simulink model "Autonomous_Driving_Car_Example1"  (R2022a)
settings: Solver=ode2  StartTime=0.0  StopTime=inf  FixedStep=1/600  RelTol=1e-3  EnableMultiTasking=on
model workspace (MAT data in the model file):
  camera_rate : Simulink.Parameter (value not decoded)
  depth_rate : Simulink.Parameter (value not decoded)
symbols that are objects in the model workspace (value not decoded): camera_rate, depth_rate
undefined symbols (not defined in the file): gcbh, height, HIL, JPEG, left, qc_get_step_size, top, Video3D, video_display_show, width
libraries: quarc_library x45, simulink x12
(part 2 of 2)

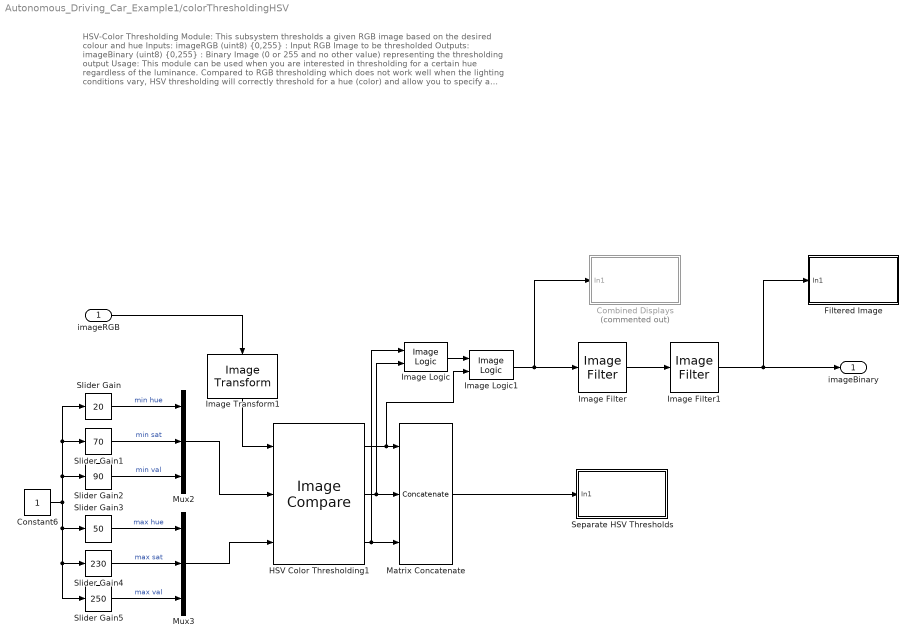
== system Autonomous_Driving_Car_Example1/colorThresholdingHSV ==
  note: HSV-Color Thresholding Module:
      |
      | This subsystem thresholds a given RGB image based on the desired colour and hue
      |
      | Inputs:
      | imageRGB (uint8) {0,255} : Input RGB Image to be thresholded
      |
      | Outputs:
      | imageBinary (uint8) {0,255} : Binary Image (0 or 255 and no other value) representing the thresholding output
      |
      | Usage:
      | This module can be used when you are interested in thresholding for a certain hue regardless of the luminance. Compared to RGB thresholding which does not work well when the lighting conditions vary, HSV thresholding will correctly threshold for a hue (color) and allow you to specify a broad range of illuminance via the saturation and value thresholds.
      |
      | The Separate HSV Thresholds display can help you tune the hue, saturation, and value separately. The final output is the logical and of the three images. The image filter sizes can be used to remove noise (Minimum) and fill holes (Maximum).
  imageRGB : Inport
  Combined Displays : Subsystem  Commented=on  LoadFcn=set_param(gcbh, 'UserData', gcb);  StartFcn=video_display_show([gcb, '/Video Display'], 'add', gcb);  mask(Video Compressed Display){algorithm=JPEG, quality=50, sample_time=-1, use_hardware=on}
      mask prompts: algorithm "Compression algorithm:"; quality "Compression quality (0-100):"; sample_time "Sample time (seconds):"; use_hardware "Use hardware acceleration for video display"
      mask help: Displays a video stream on the host, using compression to minimize bandwidth.
      mask init:
      | qc_set_display('Video\nCompressed\nDisplay');
      settings: UndoDeleteFcn=set_param(gcbh, 'UserData', gcb);  OpenFcn=video_display_show([gcb, '/Video Display'], 'show', gcb);  PreDeleteFcn=video_display_show([gcb, '/Video Display'], 'delete');
      settings: CopyFcn=|
      | set_param(gcbh, 'UserData', gcb);
      | set_param(gcbh, 'LinkStatus', 'none');
      settings: NameChangeFcn=|
      | video_display_show([get_param(gcbh, 'UserData'), '/Video Display'], 'rename', [gcb, '/Video Display']);
      | video_display_show([gcb, '/Video Display'], 'add', gcb);
      | set_param(gcbh, 'UserData', gcb);
      mask Help: web(qc_get_block_help_path(gcb));
      mask TypeOptions algorithm: Image Compress/algorithm
      mask TypeOptions quality: Image Compress/quality
      mask TypeOptions sample_time: Video Display/sample_time
      mask TypeOptions use_hardware: Video Display/use_hardware
      mask Display:
      | patch([0.98591 0.98591 0.62618 0.59072 0.56147   0.536   0.536  0.5441 0.56912 0.59207 0.60881 0.62276 0.63527 0.64364  0.6485  0.6485 0.64706 0.64499 0.63662 0.62411 0.61232 0.59837 0.58307 0.56147   0.536   0.536  0.5441  0.5747 0.60953 0.63662 0.67001  0.7034 0.72851 0.75425 0.77927 0.80294 0.82454 0.84119 0.85865 0.87395 0.88574 0.89339  0.8969 0.89969 0.89969 0.89267  0.8816 0.87044 0.85649  0.8384 0.81824 0.80294 0.78764 0.77513 0.76676 0.75776 0.76397 0.77513 0.79178 0.80987 0.82796 0.84326 0.86207 0.98528],[0.18689 0.05522 0.05522 0.05171 0.05171    0.05 0.18338 0.18338 0.19148 0.20435 0.22298 0.24863 0.28589 0.33125 0.38138 0.55139 0.59801 0.63761 0.68189 0.72149 0.74939 0.76694 0.77855 0.79367 0.79952 0.92768 0.92768 0.92768 0.92417 0.92066 0.91364  0.9032 0.89384 0.88106 0.86594 0.85073 0.82634 0.80537 0.77855 0.74363 0.70403 0.65858 0.61079 0.59099 0.41513 0.37202 0.31847 0.29048 0.25556 0.23342  0.2102 0.19382 0.18221 0.17285 0.16943 0.16124  0.1589 0.16241 0.16709 0.17168  0.1787 0.18221 0.18689 0.18689],[0.9,0.90,0.91])
      | patch([0.536 0.52601 0.46823 0.44528 0.41603 0.39101 0.35555 0.33116 0.31451 0.29291  0.2804 0.26717 0.25322 0.23999 0.22406 0.20732 0.19337 0.17528 0.15935 0.14396 0.13217 0.11759 0.10922 0.10085 0.09671 0.09392 0.09041 0.08906 0.08906 0.09464  0.0995 0.10778 0.11894 0.13145 0.14675 0.16349 0.17672 0.19409 0.20732 0.22406 0.23999 0.26159 0.27833 0.29849 0.31793 0.33602 0.35411 0.37085 0.39245 0.41603   0.536   0.536 0.53159 0.46409   0.446 0.42026 0.39587 0.37571 0.36113 0.34925 0.34088 0.33809 0.33809 0.34088 0.34583 0.35627 0.36392 0.38129 0.39587 0.41117 0.42719 0.44672  0.4676 0.48353 0.48353 0.52394   0.536],[0.05 0.04829 0.04712 0.04712 0.04829 0.05063 0.05405 0.05873 0.06107 0.06692 0.07043 0.07619 0.08087 0.08672 0.09482 0.10652 0.11696 0.13325  0.1508 0.17168 0.19499 0.22415 0.25439 0.28472 0.31379 0.35456 0.38489 0.41513 0.58055 0.63878 0.68774 0.72149 0.75641 0.78089 0.80537 0.82859 0.84029 0.85658 0.86594 0.87404  0.8834 0.89267 0.90086 0.90788 0.91247 0.91832 0.92066   0.923 0.92651 0.92768 0.92768 0.79952 0.79952 0.79952 0.79718 0.78899 0.77153 0.75056 0.72149 0.68072 0.62249  0.5549 0.41396 0.37085 0.33242 0.28121 0.25205 0.22181 0.20552 0.19499 0.18572 0.18221 0.17753 0.17636 0.17753  0.1787  0.1787],[0.9,0.90,0.91])
      | disp('Video\nCompressed\nDisplay');
  Constant6 : Constant
  Filtered Image : Subsystem  LoadFcn=set_param(gcbh, 'UserData', gcb);  StartFcn=video_display_show([gcb, '/Video Display'], 'add', gcb);  mask(Video Compressed Display){algorithm=JPEG, quality=50, sample_time=-1, use_hardware=on}
      mask prompts: algorithm "Compression algorithm:"; quality "Compression quality (0-100):"; sample_time "Sample time (seconds):"; use_hardware "Use hardware acceleration for video display"
      mask help: Displays a video stream on the host, using compression to minimize bandwidth.
      mask init:
      | qc_set_display('Video\nCompressed\nDisplay');
      settings: UndoDeleteFcn=set_param(gcbh, 'UserData', gcb);  OpenFcn=video_display_show([gcb, '/Video Display'], 'show', gcb);  PreDeleteFcn=video_display_show([gcb, '/Video Display'], 'delete');
      settings: CopyFcn=|
      | set_param(gcbh, 'UserData', gcb);
      | set_param(gcbh, 'LinkStatus', 'none');
      settings: NameChangeFcn=|
      | video_display_show([get_param(gcbh, 'UserData'), '/Video Display'], 'rename', [gcb, '/Video Display']);
      | video_display_show([gcb, '/Video Display'], 'add', gcb);
      | set_param(gcbh, 'UserData', gcb);
      mask Help: web(qc_get_block_help_path(gcb));
      mask TypeOptions algorithm: Image Compress/algorithm
      mask TypeOptions quality: Image Compress/quality
      mask TypeOptions sample_time: Video Display/sample_time
      mask TypeOptions use_hardware: Video Display/use_hardware
      mask Display:
      | patch([0.98591 0.98591 0.62618 0.59072 0.56147   0.536   0.536  0.5441 0.56912 0.59207 0.60881 0.62276 0.63527 0.64364  0.6485  0.6485 0.64706 0.64499 0.63662 0.62411 0.61232 0.59837 0.58307 0.56147   0.536   0.536  0.5441  0.5747 0.60953 0.63662 0.67001  0.7034 0.72851 0.75425 0.77927 0.80294 0.82454 0.84119 0.85865 0.87395 0.88574 0.89339  0.8969 0.89969 0.89969 0.89267  0.8816 0.87044 0.85649  0.8384 0.81824 0.80294 0.78764 0.77513 0.76676 0.75776 0.76397 0.77513 0.79178 0.80987 0.82796 0.84326 0.86207 0.98528],[0.18689 0.05522 0.05522 0.05171 0.05171    0.05 0.18338 0.18338 0.19148 0.20435 0.22298 0.24863 0.28589 0.33125 0.38138 0.55139 0.59801 0.63761 0.68189 0.72149 0.74939 0.76694 0.77855 0.79367 0.79952 0.92768 0.92768 0.92768 0.92417 0.92066 0.91364  0.9032 0.89384 0.88106 0.86594 0.85073 0.82634 0.80537 0.77855 0.74363 0.70403 0.65858 0.61079 0.59099 0.41513 0.37202 0.31847 0.29048 0.25556 0.23342  0.2102 0.19382 0.18221 0.17285 0.16943 0.16124  0.1589 0.16241 0.16709 0.17168  0.1787 0.18221 0.18689 0.18689],[0.9,0.90,0.91])
      | patch([0.536 0.52601 0.46823 0.44528 0.41603 0.39101 0.35555 0.33116 0.31451 0.29291  0.2804 0.26717 0.25322 0.23999 0.22406 0.20732 0.19337 0.17528 0.15935 0.14396 0.13217 0.11759 0.10922 0.10085 0.09671 0.09392 0.09041 0.08906 0.08906 0.09464  0.0995 0.10778 0.11894 0.13145 0.14675 0.16349 0.17672 0.19409 0.20732 0.22406 0.23999 0.26159 0.27833 0.29849 0.31793 0.33602 0.35411 0.37085 0.39245 0.41603   0.536   0.536 0.53159 0.46409   0.446 0.42026 0.39587 0.37571 0.36113 0.34925 0.34088 0.33809 0.33809 0.34088 0.34583 0.35627 0.36392 0.38129 0.39587 0.41117 0.42719 0.44672  0.4676 0.48353 0.48353 0.52394   0.536],[0.05 0.04829 0.04712 0.04712 0.04829 0.05063 0.05405 0.05873 0.06107 0.06692 0.07043 0.07619 0.08087 0.08672 0.09482 0.10652 0.11696 0.13325  0.1508 0.17168 0.19499 0.22415 0.25439 0.28472 0.31379 0.35456 0.38489 0.41513 0.58055 0.63878 0.68774 0.72149 0.75641 0.78089 0.80537 0.82859 0.84029 0.85658 0.86594 0.87404  0.8834 0.89267 0.90086 0.90788 0.91247 0.91832 0.92066   0.923 0.92651 0.92768 0.92768 0.79952 0.79952 0.79952 0.79718 0.78899 0.77153 0.75056 0.72149 0.68072 0.62249  0.5549 0.41396 0.37085 0.33242 0.28121 0.25205 0.22181 0.20552 0.19499 0.18572 0.18221 0.17753 0.17636 0.17753  0.1787  0.1787],[0.9,0.90,0.91])
      | disp('Video\nCompressed\nDisplay');
  HSV Color Thresholding1 : quarc_library/Image Processing/Generic/Image Compare  output_type=Separate planes (three HxW outputs)  source=External input ports  r_comparison=min <= pixel and pixel <= max with wrapping  r_minimum=30  r_maximum=70  g_comparison=min <= pixel and pixel <= max  g_minimum=60  g_maximum=100  b_comparison=min <= pixel and pixel <= max  b_minimum=40  b_maximum=80
      settings: SourceProductName=QUARC Targets
  Image Filter : quarc_library/Image Processing/Generic/Image Filter  filter_type=Minimum  source_of_roi=Internal dialog parameter  roi_style=[top, left, height, width]  roi=[]  maximum_roi=[]  roi_zone=Operate inside region of interest  border_type=Replicate  border_value=[0 0 0]  kernel_size=5  sigma=10  mask_size=[3 3]  kernel=int16([-2 -1 0; -1 1 1; 0 1 2])  divisor=1  offset=0  rounding=Nearest  algorithm_hint=None  threshold=100  alpha=0.9  num_frames=8  num_valid=1  gap_threshold=10  depth_threshold=255  iterations=2
      settings: AttributesFormatString=(%<filter_type>)  SourceProductName=QUARC Targets
  Image Filter1 : quarc_library/Image Processing/Generic/Image Filter  filter_type=Maximum  source_of_roi=Internal dialog parameter  roi_style=[top, left, height, width]  roi=[]  maximum_roi=[]  roi_zone=Operate inside region of interest  border_type=Replicate  border_value=[0 0 0]  kernel_size=5  sigma=10  mask_size=[7 7]  kernel=int16([-2 -1 0; -1 1 1; 0 1 2])  divisor=1  offset=0  rounding=Nearest  algorithm_hint=None  threshold=100  alpha=0.9  num_frames=8  num_valid=1  gap_threshold=10  depth_threshold=255  iterations=2
      settings: AttributesFormatString=(%<filter_type>)  SourceProductName=QUARC Targets
  Image Logic : quarc_library/Image Processing/Generic/Image Logic  algorithm=AND  source=Internal dialog parameter  row=0  column=0
      settings: AttributesFormatString=(%<algorithm>)  SourceProductName=QUARC Targets
  Image Logic1 : quarc_library/Image Processing/Generic/Image Logic  algorithm=AND  source=Internal dialog parameter  row=0  column=0
      settings: AttributesFormatString=(%<algorithm>)  SourceProductName=QUARC Targets
  Image Transform1 : quarc_library/Image Processing/Generic/Image Transform  algorithm=RGB to HSV  color_theme=KRYGCBMW  min_pixel=0  max_pixel=4000  focal_length=308  principal_point=[262 334]  radial_coeffs=[-0.3129 0.0907]  tangential_coeffs=[]  extrapolated_pixel=0  interpolation=nearest  row_coords=0  column_coords=0  output_height=480  output_width=640  angle=0  origin=[240 320]  output_origin=[240 320]  output_data_type=uint8
      settings: AttributesFormatString=(%<algorithm>)  SourceProductName=QUARC Targets
  Matrix Concatenate : Concatenate  NumInputs=3  Mode=Multidimensional array  ConcatenateDimension=2
  Mux2 : Mux  Inputs=3
  Mux3 : Mux  Inputs=3
  Separate HSV Thresholds : Subsystem  LoadFcn=set_param(gcbh, 'UserData', gcb);  StartFcn=video_display_show([gcb, '/Video Display'], 'add', gcb);  mask(Video Compressed Display){algorithm=JPEG, quality=50, sample_time=-1, use_hardware=on}
      mask prompts: algorithm "Compression algorithm:"; quality "Compression quality (0-100):"; sample_time "Sample time (seconds):"; use_hardware "Use hardware acceleration for video display"
      mask help: Displays a video stream on the host, using compression to minimize bandwidth.
      mask init:
      | qc_set_display('Video\nCompressed\nDisplay');
      settings: UndoDeleteFcn=set_param(gcbh, 'UserData', gcb);  OpenFcn=video_display_show([gcb, '/Video Display'], 'show', gcb);  PreDeleteFcn=video_display_show([gcb, '/Video Display'], 'delete');
      settings: CopyFcn=|
      | set_param(gcbh, 'UserData', gcb);
      | set_param(gcbh, 'LinkStatus', 'none');
      settings: NameChangeFcn=|
      | video_display_show([get_param(gcbh, 'UserData'), '/Video Display'], 'rename', [gcb, '/Video Display']);
      | video_display_show([gcb, '/Video Display'], 'add', gcb);
      | set_param(gcbh, 'UserData', gcb);
      mask Help: web(qc_get_block_help_path(gcb));
      mask TypeOptions algorithm: Image Compress/algorithm
      mask TypeOptions quality: Image Compress/quality
      mask TypeOptions sample_time: Video Display/sample_time
      mask TypeOptions use_hardware: Video Display/use_hardware
      mask Display:
      | patch([0.98591 0.98591 0.62618 0.59072 0.56147   0.536   0.536  0.5441 0.56912 0.59207 0.60881 0.62276 0.63527 0.64364  0.6485  0.6485 0.64706 0.64499 0.63662 0.62411 0.61232 0.59837 0.58307 0.56147   0.536   0.536  0.5441  0.5747 0.60953 0.63662 0.67001  0.7034 0.72851 0.75425 0.77927 0.80294 0.82454 0.84119 0.85865 0.87395 0.88574 0.89339  0.8969 0.89969 0.89969 0.89267  0.8816 0.87044 0.85649  0.8384 0.81824 0.80294 0.78764 0.77513 0.76676 0.75776 0.76397 0.77513 0.79178 0.80987 0.82796 0.84326 0.86207 0.98528],[0.18689 0.05522 0.05522 0.05171 0.05171    0.05 0.18338 0.18338 0.19148 0.20435 0.22298 0.24863 0.28589 0.33125 0.38138 0.55139 0.59801 0.63761 0.68189 0.72149 0.74939 0.76694 0.77855 0.79367 0.79952 0.92768 0.92768 0.92768 0.92417 0.92066 0.91364  0.9032 0.89384 0.88106 0.86594 0.85073 0.82634 0.80537 0.77855 0.74363 0.70403 0.65858 0.61079 0.59099 0.41513 0.37202 0.31847 0.29048 0.25556 0.23342  0.2102 0.19382 0.18221 0.17285 0.16943 0.16124  0.1589 0.16241 0.16709 0.17168  0.1787 0.18221 0.18689 0.18689],[0.9,0.90,0.91])
      | patch([0.536 0.52601 0.46823 0.44528 0.41603 0.39101 0.35555 0.33116 0.31451 0.29291  0.2804 0.26717 0.25322 0.23999 0.22406 0.20732 0.19337 0.17528 0.15935 0.14396 0.13217 0.11759 0.10922 0.10085 0.09671 0.09392 0.09041 0.08906 0.08906 0.09464  0.0995 0.10778 0.11894 0.13145 0.14675 0.16349 0.17672 0.19409 0.20732 0.22406 0.23999 0.26159 0.27833 0.29849 0.31793 0.33602 0.35411 0.37085 0.39245 0.41603   0.536   0.536 0.53159 0.46409   0.446 0.42026 0.39587 0.37571 0.36113 0.34925 0.34088 0.33809 0.33809 0.34088 0.34583 0.35627 0.36392 0.38129 0.39587 0.41117 0.42719 0.44672  0.4676 0.48353 0.48353 0.52394   0.536],[0.05 0.04829 0.04712 0.04712 0.04829 0.05063 0.05405 0.05873 0.06107 0.06692 0.07043 0.07619 0.08087 0.08672 0.09482 0.10652 0.11696 0.13325  0.1508 0.17168 0.19499 0.22415 0.25439 0.28472 0.31379 0.35456 0.38489 0.41513 0.58055 0.63878 0.68774 0.72149 0.75641 0.78089 0.80537 0.82859 0.84029 0.85658 0.86594 0.87404  0.8834 0.89267 0.90086 0.90788 0.91247 0.91832 0.92066   0.923 0.92651 0.92768 0.92768 0.79952 0.79952 0.79952 0.79718 0.78899 0.77153 0.75056 0.72149 0.68072 0.62249  0.5549 0.41396 0.37085 0.33242 0.28121 0.25205 0.22181 0.20552 0.19499 0.18572 0.18221 0.17753 0.17636 0.17753  0.1787  0.1787],[0.9,0.90,0.91])
      | disp('Video\nCompressed\nDisplay');
  Slider Gain : simulink/Math Operations/Slider Gain  gain=20  low=0  high=255
  Slider Gain1 : simulink/Math Operations/Slider Gain  gain=70  low=0  high=255
  Slider Gain2 : simulink/Math Operations/Slider Gain  gain=90  low=0  high=255
  Slider Gain3 : simulink/Math Operations/Slider Gain  gain=50  low=0  high=255
  Slider Gain4 : simulink/Math Operations/Slider Gain  gain=230  low=0  high=255
  Slider Gain5 : simulink/Math Operations/Slider Gain  gain=250  low=0  high=255
  imageBinary : Outport  VectorParamsAs1DForOutWhenUnconnected=off
  wires:
  HSV Color Thresholding1/3 -> Image Logic/1, Matrix Concatenate/3
  Image Logic1/1 -> Combined Displays/1(In1), Image Filter/1
  Image Logic/1 -> Image Logic1/1
  Matrix Concatenate/1 -> Separate HSV Thresholds/1(In1)
  Mux2/1 -> HSV Color Thresholding1/2
  Image Transform1/1 -> HSV Color Thresholding1/1
  Slider Gain/1 -> Mux2/1  "min hue"
  HSV Color Thresholding1/2 -> Image Logic/2, Matrix Concatenate/2
  Slider Gain5/1 -> Mux3/3  "max val"
  Slider Gain2/1 -> Mux2/3  "min val"
  Mux3/1 -> HSV Color Thresholding1/3
  Slider Gain1/1 -> Mux2/2  "min sat"
  Slider Gain4/1 -> Mux3/2  "max sat"
  HSV Color Thresholding1/1 -> Image Logic1/2, Matrix Concatenate/1
  Constant6/1 -> Slider Gain/1, Slider Gain1/1, Slider Gain2/1, Slider Gain3/1, Slider Gain5/1, Slider Gain4/1
  imageRGB/1 -> Image Transform1/1
  Slider Gain3/1 -> Mux3/1  "max hue"
  Image Filter/1 -> Image Filter1/1
  Image Filter1/1 -> Filtered Image/1(In1), imageBinary/1

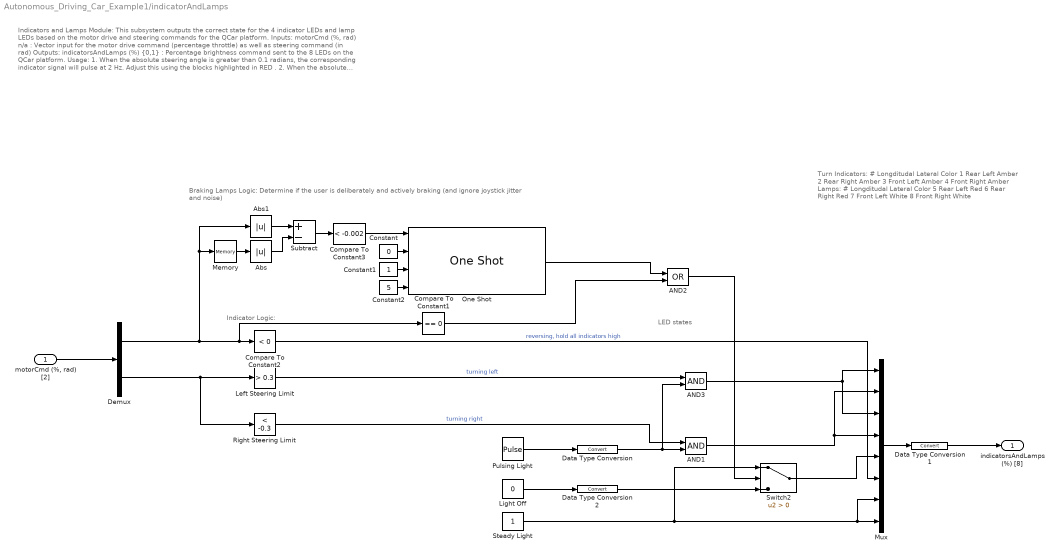
== system Autonomous_Driving_Car_Example1/indicatorAndLamps ==
  note: Indicators and Lamps Module:
      |
      | This subsystem outputs the correct state for the 4 indicator LEDs and lamp LEDs based on the motor drive and steering commands for the QCar platform.
      |
      | Inputs:
      | motorCmd (%, rad) n/a : Vector input for the motor drive command (percentage throttle) as well as steering command (in rad)
      |
      | Outputs:
      | indicatorsAndLamps (%) {0,1} : Percentage brightness command sent to the 8 LEDs on the QCar platform.
      |
      | Usage:
      | 1. When the absolute steering angle is greater than 0.1 radians, the corresponding indicator signal will pulse at 2 Hz. Adjust this using the blocks highlighted in RED .
      | 2. When the absolute motor drive command approaches 0, the brake lamps will receive 100% brightness command, and 0% brightness otherwise. Adjust this using the blocks highlighted in GREEN .
  note: Braking Lamps Logic:
      | Determine if the user is deliberately and actively braking (and ignore joystick jitter and noise)
  note: LED states
  note: Turn Indicators:
      | # Longditudal Lateral Color
      | 1 Rear Left Amber
      | 2 Rear Right Amber
      | 3 Front Left Amber
      | 4 Front Right Amber
      |
      | Lamps:
      | # Longditudal Lateral Color
      | 5 Rear Left Red
      | 6 Rear Right Red
      | 7 Front Left White
      | 8 Front Right White
  note: Indicator Logic:
  "motorCmd (%, rad) [2]" : Inport
  AND1 : Logic  IconShape=distinctive  AllPortsSameDT=off  OutDataTypeStr=boolean
  AND2 : Logic  Operator=OR  IconShape=distinctive  AllPortsSameDT=off  OutDataTypeStr=boolean
  AND3 : Logic  IconShape=distinctive  AllPortsSameDT=off  OutDataTypeStr=boolean
  Abs : Abs  SaturateOnIntegerOverflow=off
  Abs1 : Abs  SaturateOnIntegerOverflow=off
  Compare To Constant1 : simulink/Logic and Bit Operations/Compare To Constant  relop===  const=0  OutDataTypeStr=uint8
  Compare To Constant2 : simulink/Logic and Bit Operations/Compare To Constant  relop=<  const=0  OutDataTypeStr=boolean
  Compare To Constant3 : simulink/Logic and Bit Operations/Compare To Constant  relop=<  const=-0.002  OutDataTypeStr=boolean
  Constant : Constant  Value=0
  Constant1 : Constant
  Constant2 : Constant  Value=5
  Data Type Conversion : DataTypeConversion  SaturateOnIntegerOverflow=off  RndMeth=Floor
  Data Type Conversion1 : DataTypeConversion  SaturateOnIntegerOverflow=off  RndMeth=Floor
  Data Type Conversion2 : DataTypeConversion  SaturateOnIntegerOverflow=off  RndMeth=Floor
  Demux : Demux  Outputs=2
  Left Steering Limit : simulink/Logic and Bit Operations/Compare To Constant  relop=>  const=0.3  OutDataTypeStr=boolean
  Light Off : Constant  Value=0  OutDataTypeStr=boolean
  Memory : Memory
  Mux : Mux  Inputs=8
  One Shot : quarc_library/Discontinuities/One Shot  trigger_type=Falling edge  redun_pulse=Ignore extraneous pulse  width_source=External input port  pulse_width=100
      settings: SourceProductName=QUARC Targets
  Pulsing Light : DiscretePulseGenerator  Period=0.5/qc_get_step_size  PulseWidth=0.5/2/qc_get_step_size  SampleTime=qc_get_step_size
  Right Steering Limit : simulink/Logic and Bit Operations/Compare To Constant  relop=<  const=-0.3  OutDataTypeStr=boolean
  Steady Light : Constant  OutDataTypeStr=boolean
  Subtract : Sum  Inputs=+-
  Switch2 : Switch  Criteria=u2 > Threshold  SaturateOnIntegerOverflow=off  InputSameDT=off
  indicatorsAndLamps (%) [8] : Outport  VectorParamsAs1DForOutWhenUnconnected=off
  wires:
  Data Type Conversion2/1 -> Switch2/3
  Demux/2 -> Right Steering Limit/1, Left Steering Limit/1
  Light Off/1 -> Data Type Conversion2/1
  One Shot/1 -> AND2/1
  Steady Light/1 -> Mux/7, Mux/8, Switch2/1
  Compare To Constant3/1 -> One Shot/1
  Constant2/1 -> One Shot/4
  Right Steering Limit/1 -> AND1/1  "turning right"
  Mux/1 -> Data Type Conversion1/1
  Constant/1 -> One Shot/2
  Pulsing Light/1 -> Data Type Conversion/1
  Abs/1 -> Subtract/2
  Memory/1 -> Abs/1
  Abs1/1 -> Subtract/1
  Data Type Conversion/1 -> AND3/2, AND1/2
  Data Type Conversion1/1 -> indicatorsAndLamps (%) [8]/1
  Left Steering Limit/1 -> AND3/1  "turning left"
  Switch2/1 -> Mux/5
  Constant1/1 -> One Shot/3
  Demux/1 -> Compare To Constant1/1, Compare To Constant2/1, Memory/1, Abs1/1
  AND3/1 -> Mux/1, Mux/3
  "motorCmd (%, rad) [2]"/1 -> Demux/1
  Subtract/1 -> Compare To Constant3/1
  AND1/1 -> Mux/2, Mux/4
  Compare To Constant2/1 -> Mux/6  "reversing, hold all indicators high"
  Compare To Constant1/1 -> AND2/2
  AND2/1 -> Switch2/2

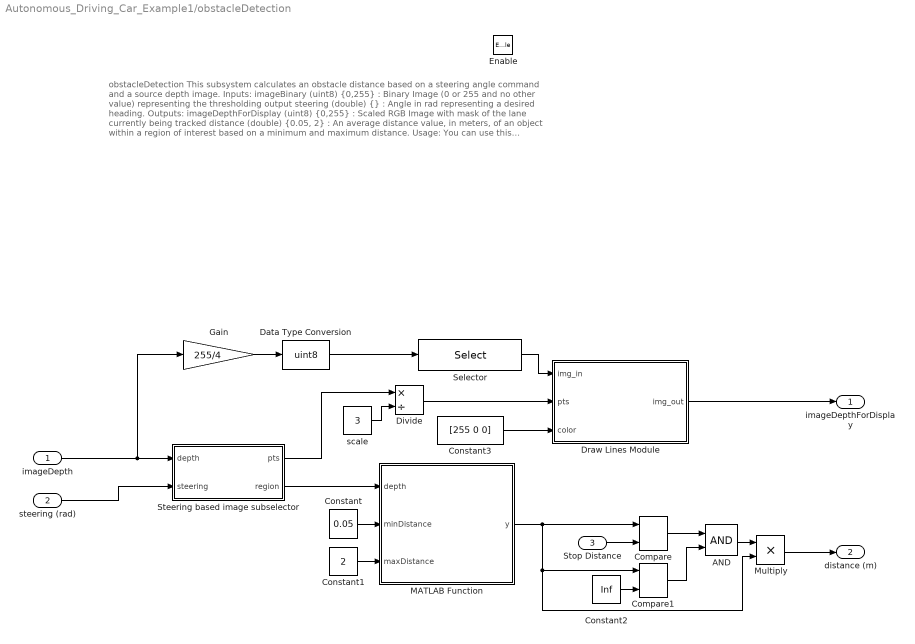
== system Autonomous_Driving_Car_Example1/obstacleDetection ==
  note: obstacleDetection
      | This subsystem calculates an obstacle distance based on a steering angle command and a source depth image.
      |
      | Inputs:
      | imageBinary (uint8) {0,255} : Binary Image (0 or 255 and no other value) representing the thresholding output
      | steering (double) {} : Angle in rad representing a desired heading.
      |
      | Outputs:
      | imageDepthForDisplay (uint8) {0,255} : Scaled RGB Image with mask of the lane currently being tracked
      | distance (double) {0.05, 2} : An average distance value, in meters, of an object within a region of interest based on a minimum and maximum distance.
      |
      | Usage:
      |
      | You can use this subsystem to determine if the desired heading angle will cause the car to colllide with an obstacle by examining the distances from a region of interest within the depth image and calculating how far the obstacle is.
  imageDepth : Inport
  steering (rad) : Inport  Port=2
  Stop Distance : Inport  Port=3
  Enable : EnablePort  PropagateVarSize=During execution
  AND : Logic  AllPortsSameDT=off  OutDataTypeStr=boolean
  Compare : quarc_library/Logic Operations/Compare  operator=>=  output_data_type=boolean
      settings: SourceProductName=QUARC Targets
  Compare1 : quarc_library/Logic Operations/Compare  operator=<  output_data_type=boolean
      settings: SourceProductName=QUARC Targets
  Constant : Constant  Value=0.05
  Constant1 : Constant  Value=2
  Constant2 : Constant  Value=Inf
  Constant3 : Constant  Value=[255 0 0]
  Data Type Conversion : DataTypeConversion  OutDataTypeStr=uint8  SaturateOnIntegerOverflow=off  RndMeth=Floor
  Divide : Product  Inputs=*/  OutDataTypeStr=Inherit: Inherit via back propagation
  Draw Lines Module : MATLAB Function  TreatAsAtomicUnit=on
  Gain : Gain  Gain=255/4
  MATLAB Function : MATLAB Function  TreatAsAtomicUnit=on
  Multiply : Product
  Selector : Selector  NumberOfDimensions=2  InputPortWidth=3  IndexOptions=Index vector (dialog),Index vector (dialog)  Indices=[1:3:360],[1:3:640]  OutputSizes=1,1
  Steering based image subselector : MATLAB Function  TreatAsAtomicUnit=on
  scale : Constant  Value=3
  imageDepthForDisplay : Outport  VectorParamsAs1DForOutWhenUnconnected=off
  distance (m) : Outport  Port=2  VectorParamsAs1DForOutWhenUnconnected=off
  wires:
  Constant3/1 -> Draw Lines Module/3(color)
  Steering based image subselector/1(pts) -> Divide/1
  Steering based image subselector/2(region) -> MATLAB Function/1(depth)
  steering (rad)/1 -> Steering based image subselector/2(steering)
  Multiply/1 -> distance (m)/1
  Constant1/1 -> MATLAB Function/3(maxDistance)
  Constant/1 -> MATLAB Function/2(minDistance)
  MATLAB Function/1(y) -> Compare/1, Multiply/2, Compare1/1
  imageDepth/1 -> Steering based image subselector/1(depth), Gain/1
  Selector/1 -> Draw Lines Module/1(img_in)
  Data Type Conversion/1 -> Selector/1
  Divide/1 -> Draw Lines Module/2(pts)
  Draw Lines Module/1(img_out) -> imageDepthForDisplay/1
  scale/1 -> Divide/2
  Gain/1 -> Data Type Conversion/1
  Stop Distance/1 -> Compare/2
  Compare/1 -> AND/1
  Compare1/1 -> AND/2
  Constant2/1 -> Compare1/2
  AND/1 -> Multiply/1

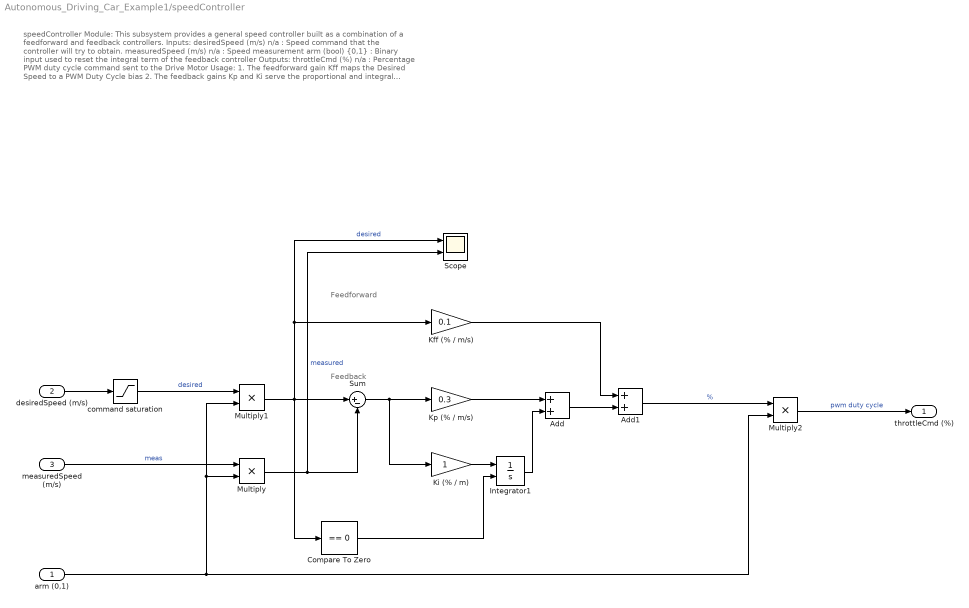
== system Autonomous_Driving_Car_Example1/speedController ==
  note: Feedforward
  note: Feedback
  note: speedController Module:
      |
      | This subsystem provides a general speed controller built as a combination of a feedforward and feedback controllers.
      |
      | Inputs:
      | desiredSpeed (m/s) n/a : Speed command that the controller will try to obtain.
      | measuredSpeed (m/s) n/a : Speed measurement
      | arm (bool) {0,1} : Binary input used to reset the integral term of the feedback controller
      |
      | Outputs:
      | throttleCmd (%) n/a : Percentage PWM duty cycle command sent to the Drive Motor
      |
      | Usage:
      | 1. The feedforward gain Kff maps the Desired Speed to a PWM Duty Cycle bias
      | 2. The feedback gains Kp and Ki serve the proportional and integral terms to output corrections to the PWM Duty Cycle so as to regulate the desired speed.
  arm (0,1) : Inport
  desiredSpeed (m/s) : Inport  Port=2
  measuredSpeed (m/s) : Inport  Port=3
  Add : Sum
  Add1 : Sum
  Compare To Zero : simulink/Logic and Bit Operations/Compare To Zero  relop===  OutDataTypeStr=boolean
  Integrator1 : Integrator  ExternalReset=either  LimitOutput=on  UpperSaturationLimit=0.4  LowerSaturationLimit=-0.4
  Kff (% / m/s) : Gain  Gain=0.1
  "Ki (% / m) " : Gain
  Kp (% / m/s) : Gain  Gain=0.3
  Multiply : Product
  Multiply1 : Product
  Multiply2 : Product
  Scope : Scope  NumInputPorts=2
  Sum : Sum  Inputs=|+-
  command saturation : Saturate  UpperLimit=5  LowerLimit=-5
  throttleCmd (%) : Outport  VectorParamsAs1DForOutWhenUnconnected=off
  wires:
  command saturation/1 -> Multiply1/1  "desired"
  arm (0,1)/1 -> Multiply1/2, Multiply/2, Multiply2/2
  measuredSpeed (m/s)/1 -> Multiply/1  "meas"
  Multiply/1 -> Sum/2, Scope/2  "measured"
  Add/1 -> Add1/2
  Add1/1 -> Multiply2/1  "%"
  Multiply1/1 -> Compare To Zero/1, Sum/1, Kff (% / m/s)/1, Scope/1  "desired"
  Integrator1/1 -> Add/2
  Multiply2/1 -> throttleCmd (%)/1  "pwm duty cycle"
  Kp (% / m/s)/1 -> Add/1
  Compare To Zero/1 -> Integrator1/2
  Kff (% / m/s)/1 -> Add1/1
  Sum/1 -> "Ki (% / m) "/1, Kp (% / m/s)/1
  "Ki (% / m) "/1 -> Integrator1/1
  desiredSpeed (m/s)/1 -> command saturation/1

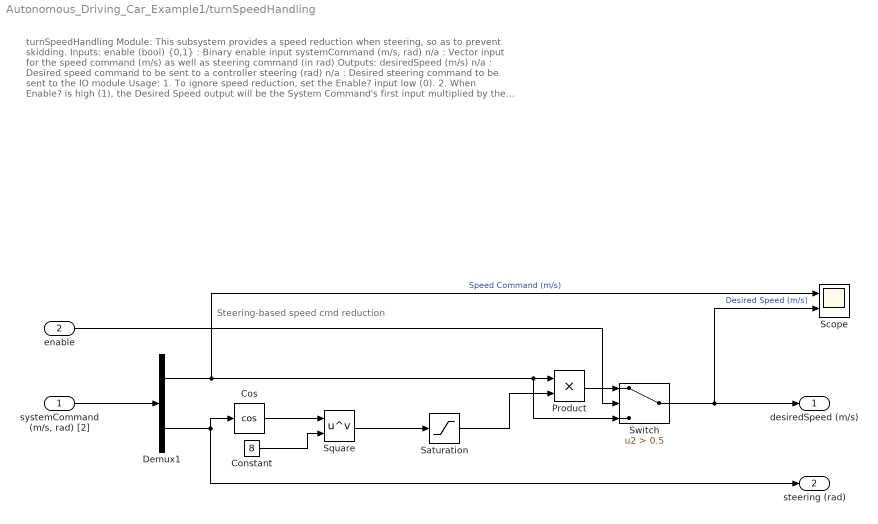
== system Autonomous_Driving_Car_Example1/turnSpeedHandling ==
  note: turnSpeedHandling Module:
      |
      | This subsystem provides a speed reduction when steering, so as to prevent skidding.
      |
      | Inputs:
      | enable (bool) {0,1} : Binary enable input
      | systemCommand (m/s, rad) n/a : Vector input for the speed command (m/s) as well as steering command (in rad)
      |
      | Outputs:
      | desiredSpeed (m/s) n/a : Desired speed command to be sent to a controller
      | steering (rad) n/a : Desired steering command to be sent to the IO module
      |
      | Usage:
      | 1. To ignore speed reduction, set the Enable? input low (0).
      | 2. When Enable? is high (1), the Desired Speed output will be the System Command's first input multiplied by the cosine of the steering. Note that the lower limit of this reduction is set to 50% of the speed command input.
  note: Steering-based speed cmd reduction
  "systemCommand (m/s, rad) [2]" : Inport
  enable : Inport  Port=2
  Constant : Constant  Value=8
  Cos : Trigonometry  Operator=cos
  Demux1 : Demux  Outputs=2
  Product : Product
  Saturation : Saturate  UpperLimit=1  LowerLimit=0.5
  Scope : Scope  NumInputPorts=2
  Square : Math  Operator=pow  SignedPower=on
  Switch : Switch  Criteria=u2 > Threshold  Threshold=0.5  SaturateOnIntegerOverflow=off  InputSameDT=off
  desiredSpeed (m/s) : Outport  VectorParamsAs1DForOutWhenUnconnected=off
  steering (rad) : Outport  Port=2  VectorParamsAs1DForOutWhenUnconnected=off
  wires:
  Cos/1 -> Square/1
  Switch/1 -> desiredSpeed (m/s)/1, Scope/2  "Desired Speed (m/s)"
  Product/1 -> Switch/1
  Saturation/1 -> Product/2
  Demux1/1 -> Product/1, Switch/3, Scope/1  "Speed Command (m/s)"
  "systemCommand (m/s, rad) [2]"/1 -> Demux1/1
  enable/1 -> Switch/2
  Constant/1 -> Square/2
  Demux1/2 -> steering (rad)/1, Cos/1
  Square/1 -> Saturation/1

== system Autonomous_Driving_Car_Example1/colorThresholdingHSV/Combined Displays ==
  In1 : Inport
  Channel : quarc_library/Signal Routing/Channel  channel=2  buffer_size=1
  Image Compress : quarc_library/Image Processing/Generic/Image Compress  algorithm=JPEG  source=Internal dialog parameter  quality=quality  output_dim=-1
  Video Display : quarc_library/Multimedia/Video Display  Tag="Autonomous_Driving_Car_Example1/colorThresholdingHSV/Combined  Displays/Video Display"  sample_time=sample_time  use_hardware=on
  wires:
  Image Compress/1 -> Channel/1
  In1/1 -> Image Compress/1
  Channel/1 -> Video Display/1

== system Autonomous_Driving_Car_Example1/colorThresholdingHSV/Filtered Image ==
  In1 : Inport
  Channel : quarc_library/Signal Routing/Channel  channel=2  buffer_size=1
  Image Compress : quarc_library/Image Processing/Generic/Image Compress  algorithm=JPEG  source=Internal dialog parameter  quality=quality  output_dim=-1
  Video Display : quarc_library/Multimedia/Video Display  Tag=Autonomous_Driving_Car_Example1/colorThresholdingHSV/Filtered Image/Video Display  sample_time=sample_time  use_hardware=on
  wires:
  Image Compress/1 -> Channel/1
  In1/1 -> Image Compress/1
  Channel/1 -> Video Display/1

== system Autonomous_Driving_Car_Example1/colorThresholdingHSV/Separate HSV Thresholds ==
  In1 : Inport
  Channel : quarc_library/Signal Routing/Channel  channel=3  buffer_size=1
  Image Compress : quarc_library/Image Processing/Generic/Image Compress  algorithm=JPEG  source=Internal dialog parameter  quality=quality  output_dim=-1
  Video Display : quarc_library/Multimedia/Video Display  Tag=Autonomous_Driving_Car_Example1/colorThresholdingHSV/Separate HSV Thresholds/Video Display  sample_time=sample_time  use_hardware=on
  wires:
  Channel/1 -> Video Display/1
  In1/1 -> Image Compress/1
  Image Compress/1 -> Channel/1

== matlab function Autonomous_Driving_Car_Example1/ROI Mask/Mask ==
  data: box input; y output
function y = fcn(box)

x_min = box(1);
x_max = box(2);
y_min = box(3);
y_max = box(4);

y = uint8(zeros(200, 820));

y(y_min:y_max, x_min:x_max) = uint8(255);

== matlab function Autonomous_Driving_Car_Example1/Lane Location/MATLAB Function ==
  data: NumberOfObjects input; u input size=2; location output; reference input
function location = fcn(NumberOfObjects, u, reference)

persistent last_location;

location = single([0; 0]);

if isempty(last_location)
    last_location = single([reference; 0]);
end

if NumberOfObjects > 0
    last_location = single([u(1); u(2)]);
end

location = last_location;

== matlab function Autonomous_Driving_Car_Example1/Diagnostics/MATLAB Function3 ==
  data: target input; y output
function y = fcn(target)


% image swaps x and y
y = [1 target(2); 
     410 target(2)];

== matlab function Autonomous_Driving_Car_Example1/Diagnostics/Draw Lines Module2 ==
  data: img_in input; img_out output; pts input; color input
function img_out = drawLines(img_in, pts, color)

% Draw lines connecting the points using the provided color

% Inputs:
% img_in    : Input RGB Image (size = m by n)
% pts       : p x-y pairs of points (px) where markers are to be drawn
% color     : 1x3 matrix of RGB color values for each marker

% Outputs:
% img_out   : Output RGB Image with the markers drawn in (size = m by n)

%% Initialization
if size(img_in, 3) == 3
    img_out = img_in;
elseif size(img_in, 3) == 1
    img_out = cat(3, img_in, img_in, img_in);
end

[p, ~] = size(pts); % determine the number of points

%% Draw the lines
    for i = 1:p-1
        % determine the max(rows_difference, col_difference) between two
        % points
        itr = max(abs(pts(i,1) - pts(i+1,1)), abs(pts(i,2) - pts(i+1,2)));
        
        % generate linear spaces of row and col values between the pts
        row_vec = round(linspace(pts(i,1), pts(i+1,1), itr));
        col_vec = round(linspace(pts(i,2), pts(i+1,2), itr));
        
        % iterate through the values and shade them right

        for j = 1:itr
            img_out(row_vec(j), col_vec(j),1) = color(1);
            img_out(row_vec(j), col_vec(j),2) = color(2);
            img_out(row_vec(j), col_vec(j),3) = color(3);
        end
    end
end

== matlab function Autonomous_Driving_Car_Example1/obstacleDetection/Draw Lines Module ==
  data: img_in input; img_out output; pts input; color input
function img_out = drawLines(img_in, pts, color)

% Draw lines connecting the points using the provided color

% Inputs:
% img_in    : Input RGB Image (size = m by n)
% pts       : p x-y pairs of points (px) where markers are to be drawn
% color     : 1x3 matrix of RGB color values for each marker

% Outputs:
% img_out   : Output RGB Image with the markers drawn in (size = m by n)

%% Initialization
if size(img_in, 3) == 3
    img_out = img_in;
elseif size(img_in, 3) == 1
    img_out = cat(3, img_in, img_in, img_in);
end

[p, ~] = size(pts); % determine the number of points

%% Draw the lines
    for i = 1:p-1
        % determine the max(rows_difference, col_difference) between two
        % points
        itr = max(abs(pts(i,1) - pts(i+1,1)), abs(pts(i,2) - pts(i+1,2)));
        
        % generate linear spaces of row and col values between the pts
        row_vec = round(linspace(pts(i,1), pts(i+1,1), itr));
        col_vec = round(linspace(pts(i,2), pts(i+1,2), itr));
        
        % iterate through the values and shade them right

        for j = 1:itr
            img_out(row_vec(j), col_vec(j),1) = color(1);
            img_out(row_vec(j), col_vec(j),2) = color(2);
            img_out(row_vec(j), col_vec(j),3) = color(3);
        end
    end
end

== matlab function Autonomous_Driving_Car_Example1/MATLAB Function ==
  data: u input; y output
function y = fcn(u)

y = u(211:410,:,:);

== matlab function Autonomous_Driving_Car_Example1/Obstacle_Avoidance ==
  data: obstacle_dist input; target_lane output; current_state output
function [target_lane, current_state] = Obstacle_Avoidance(obstacle_dist)
% Ground-Plane Clamped Obstacle Avoidance for QCar (Optimized Timing)

persistent state dist_traveled debounce_count current_cmd;
if isempty(state)
    state = 0;
    dist_traveled = 0;
    debounce_count = 0;
    current_cmd = 140;
end

% -------------------------------------------------------------
% EXECUTION BASELINE & SPEED
% -------------------------------------------------------------
dt = 0.0167;        % Effective step base
v_eff = 0.45;       % Nominal forward cruise speed (m/s)

% -------------------------------------------------------------
% DETECTION WINDOW (Clamped to prevent floor/line reflection)
% -------------------------------------------------------------
is_obstacle_ahead = (~isnan(obstacle_dist)) && ...
                    (obstacle_dist >= 0.18) && ...
                    (obstacle_dist <= 0.55);

switch state
    case 0 % ------------------- NORMAL RIGHT LANE (CRUISE) -------------------
        desired_target = 140;
        dist_traveled = 0;
        
        if is_obstacle_ahead
            debounce_count = debounce_count + 1;
            % 7 frames (~110ms): Rejects transient optical glints and shadows
            % while reacting in under 5 cm of forward vehicle motion
            if debounce_count >= 5
                state = 1;              % Initiate Left Lane Bypass
                debounce_count = 0;
                dist_traveled = 0;
            end
        else
            debounce_count = 0;
        end
        
    case 1 % ------------------- OVERTAKE (LEFT LANE) -----------------------
        desired_target = 720;
        dist_traveled = dist_traveled + v_eff * dt;
        
        % Hold passing lane for ~3.7 seconds (equivalent to ~1.65 m of physical travel):
        % • ~0.9s to shift into left lane (covers ~0.4m forward)
        % • ~1.8s to cruise past the obstacle body (covers ~0.8m forward)
        % • ~1.0s safety clearance buffer before initiating return
        if dist_traveled >= 2.8
            state = 2;                  % Begin merge back
            dist_traveled = 0;
            debounce_count = 0;
        end
        
    case 2 % ------------------- RETURNING / COOLDOWN -----------------------
        desired_target = 140;
        dist_traveled = dist_traveled + v_eff * dt;
        
        % Hold right lane for ~2.4 seconds (~1.1 m physical travel) with detector
        % locked out to prevent re-triggering on the obstacle just passed
        if dist_traveled >= 1.8
            state = 0;                  % Re-arm obstacle monitoring
            dist_traveled = 0;
            debounce_count = 0;
        end
        
    otherwise
        state = 0;
        desired_target = 140;
        dist_traveled = 0;
        debounce_count = 0;
end

% -------------------------------------------------------------
% RATE LIMITER: Smooth lateral steering slew
% -------------------------------------------------------------
% 380 px/sec: Smooth 580 px transition (140 -> 720) in exactly ~0.95 seconds
max_step = 380 * dt; 
error_step = desired_target - current_cmd;

if error_step > max_step
    current_cmd = current_cmd + max_step;
elseif error_step < -max_step
    current_cmd = current_cmd - max_step;
else
    current_cmd = desired_target;
end

target_lane = current_cmd;
current_state = state;

== matlab function Autonomous_Driving_Car_Example1/obstacleDetection/MATLAB Function ==
  data: depth input; y output; minDistance input; maxDistance input
function y = calculateDistance(depth, minDistance, maxDistance)

% This function drops depth data when outside the minDistance:maxDistance
% bounds and then averages the result. 

% u_flat = reshape(depth, 1, []);
% u_flat(u_flat < minDistance) = [];
% u_flat(u_flat > maxDistance) = [];
% y = mean(mean(u_flat));


u_flat = depth(depth <maxDistance);

u_flat  = depth(u_flat>minDistance);

y = mean(u_flat);

== matlab function Autonomous_Driving_Car_Example1/obstacleDetection/Steering based image subselector ==
  data: pts output; depth input; region output; steering input
function [pts, region] = drawBox(depth, steering)
% Input: 640 x 360
mark = 320 - (steering*260/0.5);
starting_index = mark+1-60;
region = double(depth(80:180, starting_index : starting_index + 119));
pts = [ 80, mark+1-60; 80, mark+60; 180, mark+60; 180, mark+1-60; 80, mark+1-60];

== matlab function Autonomous_Driving_Car_Example1/automatedDriving/MATLAB Function ==
  data: obstacle_distance input; speed_cmd output; stop_distance input; nominal_tracking_distance input; nominal_speed input
function speed_cmd = adaptive_cruise_control(obstacle_distance, stop_distance, nominal_tracking_distance, nominal_speed)

speed_cmd = nominal_speed;

if obstacle_distance < stop_distance
    speed_cmd = 0;
    
elseif obstacle_distance < nominal_tracking_distance
    speed_cmd = nominal_speed/(nominal_tracking_distance-stop_distance)*obstacle_distance...
              - nominal_speed/(nominal_tracking_distance-stop_distance)*stop_distance;

end

== matlab function Autonomous_Driving_Car_Example1/Diagnostics/MATLAB Function2 ==
  data: target input; y output
function y = fcn(target)


% image swaps x and y
y = [1 target; 
     410 target];

== matlab function Autonomous_Driving_Car_Example1/Diagnostics/MATLAB Function ==
  data: Binary input; y output; Color input
function y = fcn(Binary, Color)

y = Color;
[ROW, COL, ~] = size(y);

y(1:ROW, 1:COL, 1) = ((255 - Binary)/255).*Color(:,:,1) + (Binary).*Color(:, :, 1);
y(1:ROW, 1:COL, 2) = ((255 - Binary)/255).*Color(:,:,2);
y(1:ROW, 1:COL, 3) = ((255 - Binary)/255).*Color(:,:,3);

== matlab function Autonomous_Driving_Car_Example1/Diagnostics/Draw Lines Module1 ==
  data: img_in input; img_out output; pts input; color input
function img_out = drawLines(img_in, pts, color)

% Draw lines connecting the points using the provided color

% Inputs:
% img_in    : Input RGB Image (size = m by n)
% pts       : p x-y pairs of points (px) where markers are to be drawn
% color     : 1x3 matrix of RGB color values for each marker

% Outputs:
% img_out   : Output RGB Image with the markers drawn in (size = m by n)

%% Initialization
if size(img_in, 3) == 3
    img_out = img_in;
elseif size(img_in, 3) == 1
    img_out = cat(3, img_in, img_in, img_in);
end

[p, ~] = size(pts); % determine the number of points

%% Draw the lines
    for i = 1:p-1
        % determine the max(rows_difference, col_difference) between two
        % points
        itr = max(abs(pts(i,1) - pts(i+1,1)), abs(pts(i,2) - pts(i+1,2)));
        
        % generate linear spaces of row and col values between the pts
        row_vec = round(linspace(pts(i,1), pts(i+1,1), itr));
        col_vec = round(linspace(pts(i,2), pts(i+1,2), itr));
        
        % iterate through the values and shade them right

        for j = 1:itr
            img_out(row_vec(j), col_vec(j),1) = color(1);
            img_out(row_vec(j), col_vec(j),2) = color(2);
            img_out(row_vec(j), col_vec(j),3) = color(3);
        end
    end
end

== matlab function Autonomous_Driving_Car_Example1/Diagnostics/Draw Lines Module3 ==
  data: img_in input; img_out output; pts input; color input
function img_out = drawLines(img_in, pts, color)

% Draw lines connecting the points using the provided color

% Inputs:
% img_in    : Input RGB Image (size = m by n)
% pts       : p x-y pairs of points (px) where markers are to be drawn
% color     : 1x3 matrix of RGB color values for each marker

% Outputs:
% img_out   : Output RGB Image with the markers drawn in (size = m by n)

%% Initialization
if size(img_in, 3) == 3
    img_out = img_in;
elseif size(img_in, 3) == 1
    img_out = cat(3, img_in, img_in, img_in);
end

[p, ~] = size(pts); % determine the number of points

%% Draw the lines
    for i = 1:p-1
        % determine the max(rows_difference, col_difference) between two
        % points
        itr = max(abs(pts(i,1) - pts(i+1,1)), abs(pts(i,2) - pts(i+1,2)));
        
        % generate linear spaces of row and col values between the pts
        row_vec = round(linspace(pts(i,1), pts(i+1,1), itr));
        col_vec = round(linspace(pts(i,2), pts(i+1,2), itr));
        
        % iterate through the values and shade them right

        for j = 1:itr
            img_out(row_vec(j), col_vec(j),1) = color(1);
            img_out(row_vec(j), col_vec(j),2) = color(2);
            img_out(row_vec(j), col_vec(j),3) = color(3);
        end
    end
end

== matlab function Autonomous_Driving_Car_Example1/Diagnostics/MATLAB Function1 ==
  data: box input; y output
function y = fcn(box)

x_min = box(1);
x_max = box(2);
y_min = box(3);
y_max = box(4);

% image swaps x and y
y = [y_min x_min; 
     y_min x_max;
     y_max x_max;
     y_max x_min;
     y_min x_min];
